simulink model "common_pressure_testing"  (R2025a)
settings: Solver=VariableStepAuto  StartTime=0.0  StopTime=300  RelTol=1e-3
undefined symbols (not defined in the file or in its folder): National_Instruments, PCI
libraries: sldrtlib x3
settings Model: Creator=dperera  LastModifiedBy=dperera

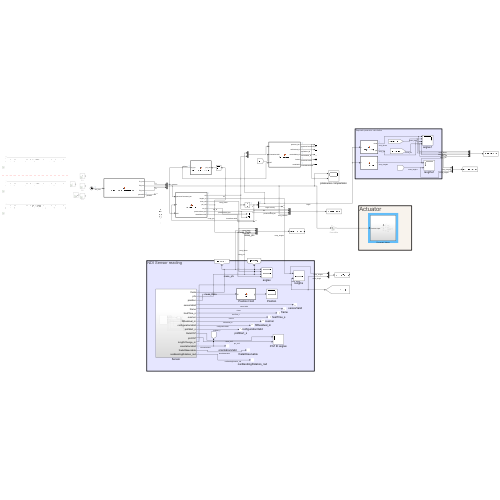
[thumbnail: Simulink's stored preview of the top-level diagram]
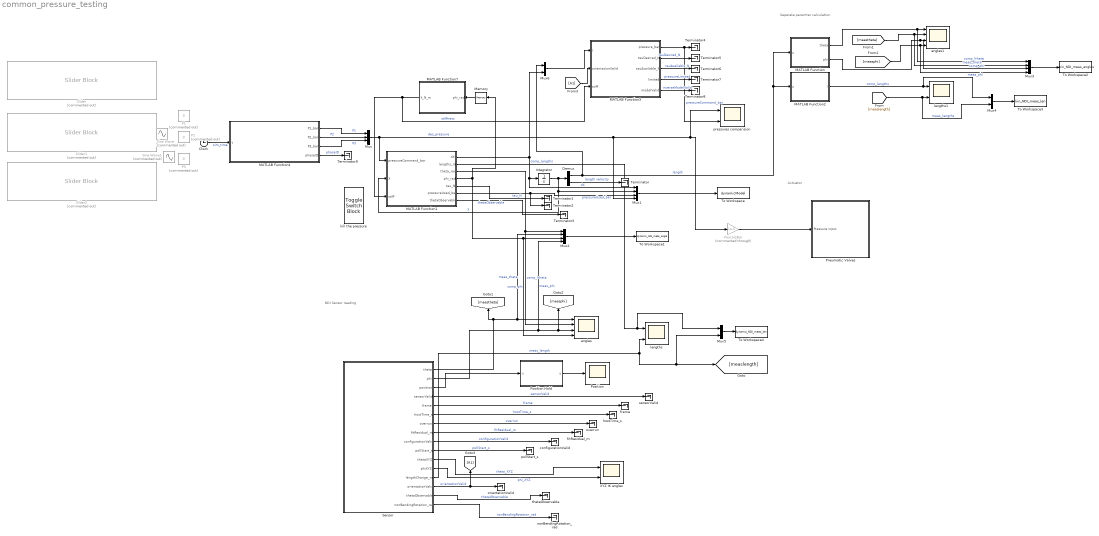
== system common_pressure_testing ==
  note: Seperate paramter calculation
  note: NDI Sensor reading
  note: Actuator
  Clock : Clock
  Demux : Demux  Outputs=2
  Integrator : Integrator  InitialCondition=[0;0;0;0]
  MATLAB Function : MATLAB Function  TreatAsAtomicUnit=on
  MATLAB Function1 : MATLAB Function  TreatAsAtomicUnit=on
  MATLAB Function2 : MATLAB Function  TreatAsAtomicUnit=on
  MATLAB Function3 : MATLAB Function  TreatAsAtomicUnit=on
  MATLAB Function4 : MATLAB Function  TreatAsAtomicUnit=on
  MATLAB Function7 : MATLAB Function  TreatAsAtomicUnit=on
  Memory : Memory  InitialCondition=0.01
  Mux : Mux  Inputs=3
  Mux1 : Mux
  Mux2 : Mux
  Mux3 : Mux
  Mux4 : Mux  Inputs=2
  Mux5 : Mux  Inputs=2
  Mux6 : Mux  Inputs=2
  P1 : Constant  Commented=on  Value=0
  P2 : Constant  Commented=on  Value=0
  P3 : Constant  Commented=on  Value=0
  Pascal2Bar : Gain  Commented=through  Gain=1e-5
  Pneumatic Valves : Subsystem
  Position : Scope
      settings: ActiveDisplayYMinimum=-0.19991149950027468  ActiveDisplayYMaximum=0.33190082979202273
  Position Hold : MATLAB Function  TreatAsAtomicUnit=on
  Sensor : Subsystem
  Sine Wave : Sin  Commented=on  Amplitude=1.5  Bias=1.5  Frequency=0.2  Phase=3*pi/2  SampleTime=0
  Sine Wave1 : Sin  Commented=on  Amplitude=1.5  Bias=1.5  Frequency=0.2  Phase=3*pi/2  SampleTime=0
  Slider : SliderBlock  Commented=on  ScaleMax=3
  Slider1 : SliderBlock  Commented=on  ScaleMax=3
  Slider2 : SliderBlock  Commented=on  ScaleMax=3
  Terminator{,1..9} (10 alike) : Terminator
  To Workspace : ToWorkspace  VariableName=dynamicModel  SaveFormat=Timeseries  SampleTime=-1
  To Workspace1 : ToWorkspace  VariableName=dynamic_NDI_meas_angle  SaveFormat=Timeseries  SampleTime=-1
  To Workspace2 : ToWorkspace  VariableName=kin_NDI_meas_angles  SaveFormat=Timeseries  SampleTime=-1
  To Workspace3 : ToWorkspace  VariableName=kin_NDI_meas_len  SaveFormat=Timeseries  SampleTime=-1
  To Workspace4 : ToWorkspace  VariableName=dynamic_NDI_meas_len  SaveFormat=Timeseries  SampleTime=-1
  XYZ IK angles : Scope  NumInputPorts=2
      settings: DataLoggingVariableName=ScopeData2
  angles : Scope  NumInputPorts=4
      settings: ActiveDisplayYMinimum=-3.9269908169872414  ActiveDisplayYMaximum=3.9269908169872414
  angles1 : Scope  NumInputPorts=4
      settings: ActiveDisplayYMinimum=-3.9269137322662839  ActiveDisplayYMaximum=3.9265599408279468  DataLoggingVariableName=ScopeData4
  configurationValid : Terminator
  fitResidual_m : Terminator
  frame : Terminator
  hostTime_s : Terminator
  kill the pressure : ToggleSwitchBlock
  lengths : Scope  NumInputPorts=2
      settings: ActiveDisplayYMinimum=-0.038844506711057027  ActiveDisplayYMaximum=0.039353697405070734  DataLoggingVariableName=ScopeData3
  lengths1 : Scope  NumInputPorts=2
      settings: ActiveDisplayYMinimum=-0.0044773637468819554  ActiveDisplayYMaximum=0.036007113704793516  DataLoggingVariableName=ScopeData5
  nonBendingRotation_rad : Terminator
  orientationValid : Terminator
  overrun : Terminator
  pollStart_s : Terminator
  pressures comparision : Scope  NumInputPorts=2
      settings: ActiveDisplayYMinimum=-0.37499998444395971  ActiveDisplayYMaximum=3.3749998599956381  DataLoggingVariableName=ScopeData6
  sensorValid : Terminator
  thetaObservable : Terminator
  wires:
  Pascal2Bar/1 -> Pneumatic Valves/1(Pressure input)
  Sensor/6(hostTime_s) -> hostTime_s/1  "hostTime_s"
  Sensor/2(phi) -> Mux2/4, angles/3, [measphi]  "meas_phi"
  Sensor/10(pollStart_s) -> pollStart_s/1  "pollStart_s"
  Sensor/9(configurationValid) -> configurationValid/1  "configurationValid"
  Sensor/3(position) -> Position Hold/1(u)
  Sensor/7(overrun) -> overrun/1  "overrun"
  Sensor/11(thetaXYZ) -> XYZ IK angles/1  "theta_XYZ"
  Sensor/4(sensorValid) -> sensorValid/1  "sensorValid"
  Sensor/12(phiXYZ) -> XYZ IK angles/2  "phi_XYZ"
  Sensor/5(frame) -> frame/1  "frame"
  Sensor/8(fitResidual_m) -> fitResidual_m/1  "fitResidual_m"
  Position Hold/1(y) -> Position/1
  Sensor/1(theta) -> Mux2/2, angles/1, [meastheta]  "meas_theta"
  Sensor/13(lengthChange_m) -> lengths/2, Mux5/2, [measlength]  "meas_length"
  Sensor/15(thetaObservable) -> thetaObservable/1  "thetaObservable"
  Sensor/14(orientationValid) -> [A1], orientationValid/1  "orientationValid"
  Sensor/16(nonBendingRotation_rad) -> nonBendingRotation_rad/1  "nonBendingRotation_rad"
  Mux/1 -> Mux1/4, pressures comparision/1, Pascal2Bar/1, MATLAB Function1/1(pressureCommand_bar)  "des_pressure"
  MATLAB Function4/1(P1_bar) -> Mux/1  "P1"
  MATLAB Function4/2(P2_bar) -> Mux/2  "P2"
  MATLAB Function4/3(P3_bar) -> Mux/3  "P3"
  MATLAB Function1/1(dX) -> Mux6/2, Mux1/1, Integrator/1  "dX"
  Integrator/1 -> MATLAB Function1/2(X), Mux1/2, Demux/1  "X"
  Demux/2 -> Terminator/1  "length velocity"
  MATLAB Function1/3(theta_rad) -> angles/2, Mux2/1  "comp_ltheta"
  MATLAB Function1/4(phi_rad) -> angles/4, Mux2/3, Memory/1  "comp_phi"
  MATLAB Function1/2(lengths_m) -> Mux5/1, lengths/1  "comp_lengths"
  Demux/1 -> Mux6/1, MATLAB Function2/1(u), MATLAB Function/1(u)  "length"
  MATLAB Function/1(theta) -> Mux3/1, angles1/1  "comp_ltheta"
  MATLAB Function/2(phi) -> Mux3/3, angles1/3  "comp_phi"
  MATLAB Function2/1(l) -> Mux4/1, lengths1/1  "comp_lengths"
  [measlength] -> Mux4/2, lengths1/2  "meas_lengths"
  [meastheta] -> Mux3/2, angles1/2  "meas_theta"
  [measphi] -> Mux3/4, angles1/4  "meas_phi"
  MATLAB Function1/5(tau_N) -> Terminator1/1  "tau_N"
  MATLAB Function1/6(pressureUsed_bar) -> Terminator2/1, Mux1/3  "pressureUsed_bar"
  MATLAB Function1/7(thetaObservable) -> Terminator3/1  "thetaObservable"
  Mux1/1 -> To Workspace/1
  Mux2/1 -> To Workspace1/1
  Mux3/1 -> To Workspace2/1
  Mux4/1 -> To Workspace3/1
  Mux5/1 -> To Workspace4/1
  Mux6/1 -> MATLAB Function3/1(l)
  [A1] -> MATLAB Function3/2(orientationValid)
  MATLAB Function3/1(pressure_bar) -> pressures comparision/2, Terminator4/1  "pressureCommand_bar"
  MATLAB Function3/2(tauDesired_N) -> Terminator5/1  "tauDesired_N"
  MATLAB Function3/3(tauAvailable_N) -> Terminator6/1  "tauAvailable_N"
  MATLAB Function3/4(limited) -> Terminator7/1  "pressureLimited"
  MATLAB Function3/5(modelValid) -> Terminator8/1  "inverseModelValid"
  MATLAB Function7/1(k_N_m) -> MATLAB Function3/3(stiff), MATLAB Function1/3(stiff)  "stiffness"
  Memory/1 -> MATLAB Function7/1(phi_rad)
  Clock/1 -> MATLAB Function4/1(t)  "sim_time"
  MATLAB Function4/4(phaseID) -> Terminator9/1  "phaseID"

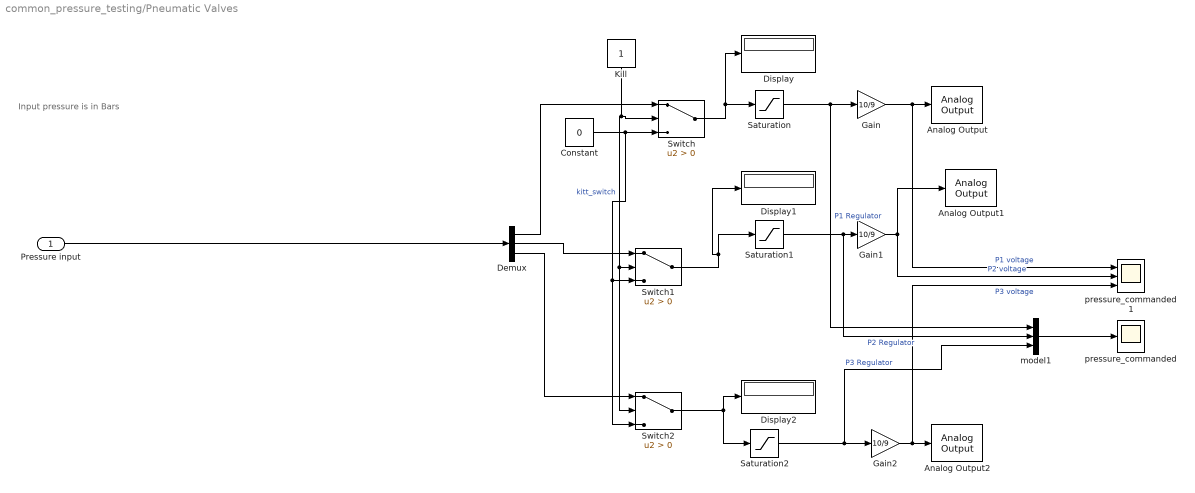
== system common_pressure_testing/Pneumatic Valves ==
  note: Input pressure is in Bars
  Pressure input : Inport
  Analog Output : sldrtlib/Analog Output  SampleTime=1/100  MaxMissedTicks=inf  ShowMissedTicks=off  YieldWhenWaiting=off  DrvName=National_Instruments/PCI-6703  DrvAddress=4294967295  DrvOptions=0  Channels=1  RangeMode=1  VoltRange=1  InitialValue=0  FinalValue=0
      settings: AttributesFormatString=National Instruments\nPCI-6703 [auto]
  Analog Output1 : sldrtlib/Analog Output  SampleTime=1/100  MaxMissedTicks=inf  ShowMissedTicks=off  YieldWhenWaiting=off  DrvName=National_Instruments/PCI-6703  DrvAddress=4294967295  DrvOptions=0  Channels=2  RangeMode=1  VoltRange=1  InitialValue=0  FinalValue=0
      settings: AttributesFormatString=National Instruments\nPCI-6703 [auto]
  Analog Output2 : sldrtlib/Analog Output  SampleTime=1/100  MaxMissedTicks=inf  ShowMissedTicks=off  YieldWhenWaiting=off  DrvName=National_Instruments/PCI-6703  DrvAddress=4294967295  DrvOptions=0  Channels=3  RangeMode=1  VoltRange=1  InitialValue=0  FinalValue=0
      settings: AttributesFormatString=National Instruments\nPCI-6703 [auto]
  Constant : Constant  Value=0
  Demux : Demux  Outputs=3
  Display : Display
  Display1 : Display
  Display2 : Display
  Gain : Gain  Gain=10/9
  Gain1 : Gain  Gain=10/9
  Gain2 : Gain  Gain=10/9
  Kill : Constant
  Saturation : Saturate  UpperLimit=3  LowerLimit=0
  Saturation1 : Saturate  UpperLimit=3  LowerLimit=0
  Saturation2 : Saturate  UpperLimit=3  LowerLimit=0
  Switch : Switch  Criteria=u2 > Threshold  SaturateOnIntegerOverflow=off  InputSameDT=off
  Switch1 : Switch  Criteria=u2 > Threshold  SaturateOnIntegerOverflow=off  InputSameDT=off
  Switch2 : Switch  Criteria=u2 > Threshold  SaturateOnIntegerOverflow=off  InputSameDT=off
  model1 : Mux  Inputs=3
  pressure_commanded : Scope
      settings: ActiveDisplayYMinimum=-0.37499998444395971  ActiveDisplayYMaximum=3.3749998599956381  DataLoggingVariableName=ScopeData7
  pressure_commanded1 : Scope  NumInputPorts=3
      settings: ActiveDisplayYMinimum=2.6976716839134527  ActiveDisplayYMaximum=3.13423095014111  DataLoggingVariableName=ScopeData8
  wires:
  Constant/1 -> Switch2/3, Switch1/3, Switch/3
  Kill/1 -> Switch2/2, Switch1/2, Switch/2  "kitt_switch"
  Switch/1 -> Display/1, Saturation/1
  Gain/1 -> pressure_commanded1/1, Analog Output/1  "P1 voltage"
  Saturation/1 -> model1/1, Gain/1  "P1 Regulator"
  Demux/3 -> Switch2/1
  Gain1/1 -> pressure_commanded1/2, Analog Output1/1  "P2 voltage"
  Gain2/1 -> pressure_commanded1/3, Analog Output2/1  "P3 voltage"
  Saturation2/1 -> model1/3, Gain2/1  "P3 Regulator"
  Switch2/1 -> Saturation2/1, Display2/1
  Demux/2 -> Switch1/1
  Switch1/1 -> Saturation1/1, Display1/1
  model1/1 -> pressure_commanded/1
  Saturation1/1 -> model1/2, Gain1/1  "P2 Regulator"
  Demux/1 -> Switch/1
  Pressure input/1 -> Demux/1

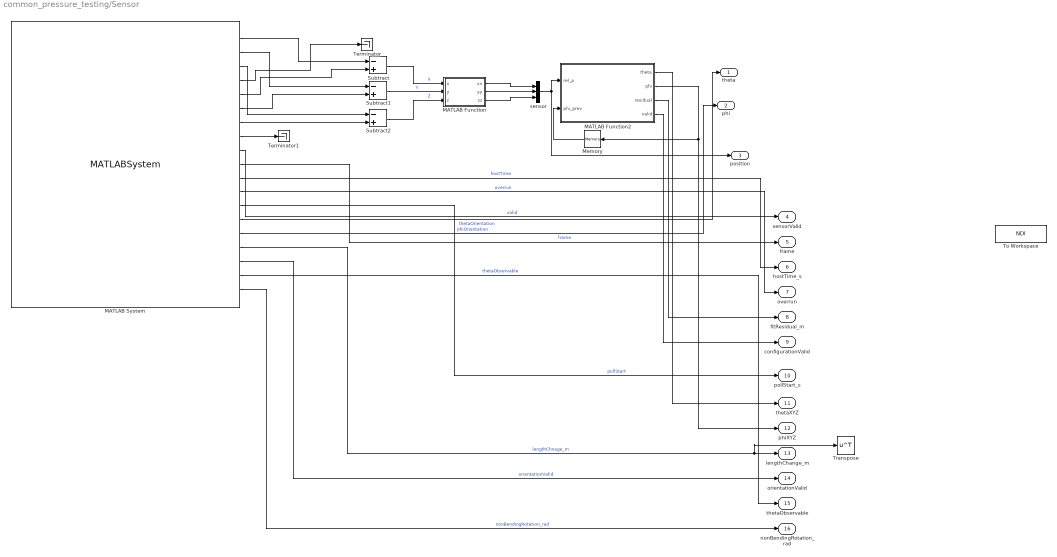
== system common_pressure_testing/Sensor ==
  MATLAB Function : MATLAB Function  TreatAsAtomicUnit=on
  MATLAB Function2 : MATLAB Function  TreatAsAtomicUnit=on
  MATLAB System : MATLABSystem  System=AuroraReader_s2_Position_only  Port=COM12  BaudRate=ndiConfig.BaudRate  SamplePeriod=ndiConfig.SamplePeriod  BaseSensorId=0A  TipSensorId=0B  CalibrationFile=C:\Users\dperera\OneDrive - Texas A&M University\Lab\Research\fDyn_ExpCom\hyDyn_Ctrl\ndi_orientation_recordings\calibration_20260930_190505_898.mat  PreflightSeconds=5  ActuatorRadius=0.013  SimulateUsing=Interpreted execution
      mask Type: AuroraReader_s2_Position_only
  Memory : Memory  InitialCondition=0.0001
  Subtract : Sum  Inputs=-+
  Subtract1 : Sum  Inputs=-+
  Subtract2 : Sum  Inputs=-+
  Terminator : Terminator
  Terminator1 : Terminator
  To Workspace : ToWorkspace  VariableName=NDI  SaveFormat=Timeseries  SampleTime=-1
  Transpose : Math  Operator=transpose
  sensor : Mux  Inputs=3
  theta : Outport
  phi : Outport  Port=2
  position : Outport  Port=3
  sensorValid : Outport  Port=4
  frame : Outport  Port=5
  hostTime_s : Outport  Port=6
  overrun : Outport  Port=7
  fitResidual_m : Outport  Port=8
  configurationValid : Outport  Port=9
  pollStart_s : Outport  Port=10
  thetaXYZ : Outport  Port=11
  phiXYZ : Outport  Port=12
  lengthChange_m : Outport  Port=13
  orientationValid : Outport  Port=14
  thetaObservable : Outport  Port=15
  nonBendingRotation_rad : Outport  Port=16
  wires:
  MATLAB System/2 -> Subtract1/1
  MATLAB Function/3(zz) -> sensor/3
  Subtract1/1 -> MATLAB Function/2(y)  "Y"
  Subtract2/1 -> MATLAB Function/3(z)  "Z"
  MATLAB System/5 -> Subtract/2
  sensor/1 -> position/1, MATLAB Function2/1(rel_p)
  MATLAB System/8 -> Terminator1/1
  MATLAB Function/1(xx) -> sensor/1
  Subtract/1 -> MATLAB Function/1(x)  "X"
  MATLAB Function/2(yy) -> sensor/2
  MATLAB System/1 -> Subtract/1
  MATLAB Function2/2(phi) -> Memory/1, phiXYZ/1
  MATLAB System/7 -> Subtract2/2
  MATLAB System/4 -> Terminator/1
  MATLAB System/3 -> Subtract2/1
  MATLAB System/6 -> Subtract1/2
  Memory/1 -> MATLAB Function2/2(phi_prev)
  MATLAB System/9 -> sensorValid/1  "valid"
  MATLAB System/11 -> hostTime_s/1  "hostTime"
  MATLAB System/12 -> overrun/1  "overrun"
  MATLAB Function2/3(residual) -> fitResidual_m/1
  MATLAB Function2/4(valid) -> configurationValid/1
  MATLAB System/13 -> pollStart_s/1  "pollStart"
  MATLAB System/14 -> theta/1  "thetaOrientation"
  MATLAB System/15 -> phi/1  "phiOrientation"
  MATLAB Function2/1(theta) -> thetaXYZ/1
  MATLAB System/16 -> Transpose/1, lengthChange_m/1  "lengthChnage_m"
  MATLAB System/17 -> orientationValid/1  "orientationValid"
  MATLAB System/18 -> thetaObservable/1  "thetaObservable"
  MATLAB System/19 -> nonBendingRotation_rad/1  "nonBendingRotation_rad"
  MATLAB System/10 -> frame/1  "frame"

== matlab function common_pressure_testing/MATLAB Function7 ==
  data: phi_rad input; k_N_m output
function k_N_m = stiffnessFromPhiBlock(phi_rad)
%#codegen
% Scalar P1 effective stiffness from the 2026-10-02 fitted data (N/m).
% Input may be current phi or externally delayed phi, in radians.
% Endpoint extension: <=0.09425 rad -> 4132; >=2.05594 rad -> 953.333.
% Invalid input uses the near-straight endpoint (not a sensor-validity gate).
breaks = [0.094252336020426999 0.31719551885716302 ...
          0.84254655402063705 1.3628983100343199 ...
          1.7568402609821301 2.0559364288348001];
coefs = [-301.18295127845971 -90.779050026315701 -3508.295263988015 4132; ...
          8648.306884889811 -4672.8276757423591 -3593.6820922138418 3342; ...
          222.76060985869111 882.71017208803505 -1342.7968944369923 1418.3333333333301; ...
          341.14621515352195 107.09908322703643 -243.20935379879649 990; ...
          254.06580436465293 166.20780898136815 0 931.66666666666697];
if ~isfinite(phi_rad) || phi_rad <= breaks(1)
    k_N_m = 4132;
    return;
end
if phi_rad >= breaks(6)
    k_N_m = 953.333333333333;
    return;
end
segment = 1;
for j = 2:5
    if phi_rad >= breaks(j), segment = j; end
end
x = phi_rad-breaks(segment);
k_N_m = ((coefs(segment,1)*x+coefs(segment,2))*x ...
           +coefs(segment,3))*x+coefs(segment,4);
end

== matlab function common_pressure_testing/MATLAB Function1 ==
  data: pressureCommand_bar input; X input; dX output; lengths_m output; theta_rad output; phi_rad output; tau_N output; pressureUsed_bar output; thetaObservable output; stiff input
% function dX  = DynamicModel(p, X)
%#codegen
% This file computes length velocity and accelration from pressures using the dynamic model.
%
% Inputs:
%   p   : pressures [3x1] (Pa)
%   X   : length derivatives [4x1] (m)
%         [l2; l3; dl2; dl3]
%
% Output:
%   dX  : length derivatives [4x1] (m)
%         [dl2; dl3; ddl2; ddl3]

function [dX, lengths_m, theta_rad, phi_rad, tau_N, ...
          pressureUsed_bar, thetaObservable] = forwardModel(pressureCommand_bar, X, stiff)
%#codegen
% pressureCommand_bar = [P1; P2; P3], nonnegative bar
% X = [l2; l3; dl2; dl3], with l1 = -l2-l3

L = 0.17411;
r = 0.013; % PMA radial offset from backbone (m)
mass = 0.1;
K = 650 * [2 1; 1 2];
% K = stiff * [2 1; 1 2];
D = 40 * eye(2);
gArm = [0; 0; -9.81];
mu = 2000;
lengthBounds = [-0.035; 0.035; 1e6];

% pressureUsed_bar = min(max(pressureCommand_bar, 0), 3);
pressureUsed_bar = max(min(max(pressureCommand_bar, 0), 3) - 0.8, 0);

pressureDiameter_m = 0.013; % Effective pressure-area diameter, independent of r
pressureRadius_m = pressureDiameter_m/2;
area = pi * pressureRadius_m^2;

% Positive P1, P2, P3 give the established -X, -60°, +60°
% nominal bending directions, respectively.
tau_N = area * 1e5 * [-1 1 0; -1 0 1] * pressureUsed_bar;

dX = armS_single_entry(0, X, L, r, mass, gArm, ...
                       K, D, tau_N, mu, lengthBounds);

l2 = X(1);
l3 = X(2);
lengths_m = [-l2-l3; l2; l3];

u = (l2+l3)/r;
v = (l3-l2)/(sqrt(3)*r);
phi_rad = hypot(u, v);
theta_rad = atan2(v, u);
thetaObservable = phi_rad > 0.5*pi/180;


end

== matlab function common_pressure_testing/MATLAB Function ==
  data: u input; theta output; phi output
function [theta, phi] = length2config(u)
%#codegen
% This file convert the length changes into theta/phi
%
% Inputs:
%   u       : length change[2x1] (m)
%             [l2; l3]
%
% Outputs:
%   theta   : bending direction [constant] (rad)
%   phi     : bending amount [constant] (rad)

l = [0.0; u(1); u(2)];
r  = 0.013;

c = [atan2(l(3) - l(2), sqrt(0.3e1) * (l(2) + l(3)));
    0.2e1 / 0.3e1 / r * sqrt((3 * l(2) ^ 2 + 3 * l(3) * l(2) + 3 * l(3) ^ 2))];

theta = c(1);
phi = c(2);

end

== matlab function common_pressure_testing/MATLAB Function2 ==
  data: u input; l output
function l = lengthVector(u)
%#codegen
% This file create the length vector
%
% Inputs:
%   u       : length change[2x1] (m)
%             [l2; l3]
%
% Outputs:
%   l   : bending direction [3x1] (m)

l = [-(u(1) + u(2)); u(1); u(2)];

end

== matlab function common_pressure_testing/Position Hold ==
  data: u input; y output
function y = fcn(u)
persistent lastPosition
if isempty(lastPosition), lastPosition=nan(3,1); end
if all(isfinite(u)), lastPosition=u; end
y=lastPosition;
end

== matlab function common_pressure_testing/Sensor/MATLAB Function ==
  data: x input; xx output; y input; z input; yy output; zz output
function [xx,yy,zz] = rotateX90(x,y,z)

    R = [1 0 0;
         0 0 1;
         0 -1 0];

    p = R*[x;y;z]*0.001;

    xx=p(1);
    yy=p(2);
    zz=p(3);

    
end

== matlab function common_pressure_testing/Sensor/MATLAB Function2 ==
  data: rel_p input; theta output; phi output; phi_prev input; residual output; valid output
function [theta,phi,residual,valid] = xyz2ThetaPhi(rel_p,phi_prev)
persistent lastPhi lastTheta lastOutputTheta lastOutputPhi lastResidual
if isempty(lastPhi)
    lastPhi=0.0001; lastTheta=0;
    lastOutputTheta=NaN; lastOutputPhi=NaN; lastResidual=NaN;
end
% Keep the external memory for compatibility; never use its NaN.
if isfinite(phi_prev), lastPhi=phi_prev; end
[theta,phi,residual,valid]=ndiSupportFnc.configuration(rel_p,lastPhi,lastTheta);
if valid
    lastPhi=phi; lastTheta=theta;
    lastOutputTheta=theta; lastOutputPhi=phi; lastResidual=residual;
else
    % Scope outputs hold, but configurationValid remains false.
    theta=lastOutputTheta; phi=lastOutputPhi; residual=lastResidual;
end
end

== matlab function common_pressure_testing/MATLAB Function3 ==
  data: l input; pressure_bar output; tauDesired_N output; tauAvailable_N output; limited output; modelValid output; orientationValid input; stiff input
function [pressure_bar, tauDesired_N, tauAvailable_N, limited, modelValid] = inverseModel(l, orientationValid, stiff)
%#codegen
% measured = [l2;l3;dl2;dl3;ddl2;ddl3] in SI units.
% Nonnegative pressure mapping uses the smallest common P1 pressure.

pressure_bar = zeros(3,1);
tauDesired_N = zeros(2,1);
tauAvailable_N = zeros(2,1);
limited = false;
modelValid = false;
if ~orientationValid || ~all(isfinite(l))
    return;
end
q = l(1:2);
dq = l(3:4);
ddq = l(5:6);
params.N = 1;
params.L = 0.17411;
params.r = 0.013;
params.mi = 0.1;
params.g = [0;0;-9.81];
params.K = 650*[2 1;1 2];
% params.K = stiff * [2 1; 1 2];
params.D = 40*eye(2);
params.mu = 2000;
params.lKbounds = [-0.035;0.035;1e6];
[M,C,G] = armS_single_core(q,dq,params);
Keff = params.K;
for i = 1:2
    Keff(i,i) = Keff(i,i) + 0.5*params.lKbounds(3)*(2 + ...
        tanh(params.mu*(q(i)-params.lKbounds(2))) - ...
        tanh(params.mu*(q(i)-params.lKbounds(1))));
end
tauDesired_N = M*ddq + (C+params.D)*dq + G + Keff*q;
if ~all(isfinite(tauDesired_N))
    tauDesired_N = zeros(2,1);
    return;
end
forcePerBar = pi*(params.r/2)^2*1e5;
forceBar = tauDesired_N/forcePerBar;
p1 = max([0;-forceBar(1);-forceBar(2)]);
effective = max([p1;p1+forceBar(1);p1+forceBar(2)],0);
deadzone_bar = 0.8;
maxCommand_bar = 3.0;
maxEffective_bar = maxCommand_bar-deadzone_bar;
peak = max(effective);
if peak > maxEffective_bar
    effective = effective*(maxEffective_bar/peak);
    limited = true;
end
for i = 1:3
    if effective(i) > 1e-8
        pressure_bar(i) = effective(i)+deadzone_bar;
    end
end
tauAvailable_N = forcePerBar*[-1 1 0;-1 0 1]*effective;
modelValid = true;
end

== matlab function common_pressure_testing/MATLAB Function4 ==
  data: t input; P1_bar output; P2_bar output; P3_bar output; phaseID output
function [P1_bar, P2_bar, P3_bar, phaseID] = commonPressureSequenceBlock(t)
%#codegen
% t is simulation time in seconds from a Clock block.
% Columns: target common pressure, target differential, ramp time, hold time.
% Positive differential gives P2 = P3 > P1.

schedule = [ ...
    0.0,  0.0, 0, 10; ...  % 1: zero reference
    1.2,  0.0, 5, 15; ...  % 2-6: common 1.2 bar
    1.2,  0.2, 5, 15; ...
    1.2,  0.0, 5, 10; ...
    1.2, -0.2, 5, 15; ...
    1.2,  0.0, 5, 10; ...
    1.6,  0.0, 5, 15; ...  % 7-11: common 1.6 bar
    1.6,  0.2, 5, 15; ...
    1.6,  0.0, 5, 10; ...
    1.6, -0.2, 5, 15; ...
    1.6,  0.0, 5, 10; ...
    2.0,  0.0, 5, 15; ...  % 12-16: common 2.0 bar
    2.0,  0.2, 5, 15; ...
    2.0,  0.0, 5, 10; ...
    2.0, -0.2, 5, 15; ...
    2.0,  0.0, 5, 10; ...
    0.0,  0.0, 5, 15];     % 17: return to zero

P1_bar = 0.0;
P2_bar = 0.0;
P3_bar = 0.0;
phaseID = 0.0;
if ~isfinite(t) || t < 0.0
    return;
end

elapsed = 0.0;
previousCommon = 0.0;
previousDifferential = 0.0;
common = 0.0;
differential = 0.0;

for k = 1:size(schedule, 1)
    targetCommon = schedule(k, 1);
    targetDifferential = schedule(k, 2);
    rampSeconds = schedule(k, 3);
    holdSeconds = schedule(k, 4);

    if rampSeconds > 0.0 && t < elapsed + rampSeconds
        fraction = (t - elapsed)/rampSeconds;
        blend = fraction*fraction*(3.0 - 2.0*fraction);
        common = previousCommon + blend*(targetCommon - previousCommon);
        differential = previousDifferential + ...
            blend*(targetDifferential - previousDifferential);
        phaseID = double(k);
        break;
    end
    elapsed = elapsed + rampSeconds;

    if t < elapsed + holdSeconds
        common = targetCommon;
        differential = targetDifferential;
        phaseID = double(k);
        break;
    end
    elapsed = elapsed + holdSeconds;
    previousCommon = targetCommon;
    previousDifferential = targetDifferential;
end

% Preserve mean pressure and set P2-P1 = P3-P1 = differential.
P1_bar = common - (2.0/3.0)*differential;
P2_bar = common + (1.0/3.0)*differential;
P3_bar = P2_bar;

P1_bar = min(max(P1_bar, 0.0), 3.0);
P2_bar = min(max(P2_bar, 0.0), 3.0);
P3_bar = min(max(P3_bar, 0.0), 3.0);
end
